simulink model "StampFly_IMU400"  (R2026b)
settings: Solver=FixedStepDiscrete  StopTime=inf  FixedStep=Official.Step
PostLoadFcn:
  | run(fullfile(fileparts(get_param('StampFly_IMU400','FileName')),'config','startup.m'));
InitFcn:
  | init_imu_flight;
undefined symbols (not defined in the file): Bottom, Official
libraries: slpidlib x7, simulink x4, mspfiltlib x1
(part 3 of 4)

== system StampFly_IMU400/SensorCorrection400/VerticalAcceleration/VerticalLowpass ==
  Input : Inport
  Dt : Inport  Port=2
  Reset : Inport  Port=3
  Enable : Inport  Port=4
  Denominator : Sum
  InputTerm : Product  Inputs=*/
  InputTimesDt : Product  Inputs=**
  PreviousFiltered : UnitDelay  InitialCondition=single(0)  SampleTime=.0025
  PreviousTerm : Product  Inputs=*/
  PreviousTimesT : Product  Inputs=**
  ResetPrevious : Switch  Criteria=u2 ~= 0  SaturateOnIntegerOverflow=off  InputSameDT=off
  TimeConstantS : Constant  Value=single(0.10000000000000001)
  UpdateOrHold : Switch  Criteria=u2 ~= 0  SaturateOnIntegerOverflow=off  InputSameDT=off
  UpdatedFiltered : Sum
  ZeroOnReset : Constant  Value=single(0)
  Filtered : Outport
  wires:
  Input/1 -> InputTimesDt/1
  Denominator/1 -> PreviousTerm/2, InputTerm/2
  InputTimesDt/1 -> InputTerm/1
  Dt/1 -> Denominator/2, InputTimesDt/2
  TimeConstantS/1 -> PreviousTimesT/2, Denominator/1
  Enable/1 -> UpdateOrHold/2
  InputTerm/1 -> UpdatedFiltered/2
  UpdatedFiltered/1 -> UpdateOrHold/1
  UpdateOrHold/1 -> PreviousFiltered/1, Filtered/1
  ZeroOnReset/1 -> ResetPrevious/1
  Reset/1 -> ResetPrevious/2
  PreviousFiltered/1 -> ResetPrevious/3
  ResetPrevious/1 -> UpdateOrHold/3, PreviousTimesT/1
  PreviousTimesT/1 -> PreviousTerm/1
  PreviousTerm/1 -> UpdatedFiltered/1

== system StampFly_IMU400/AttitudeAltitudeEstimation400/IMUAttitude400/FusionState/UpdateWhenReady ==
  Accel : Inport  PortDimensions=[1 3]
  Gyro : Inport  Port=2  PortDimensions=[1 3]
  Reset : ResetPort  DisableCoverage=on  ResetTriggerType=level
  IMU Filter : mspfiltlib/IMU Filter  DispRefFrame=NED  OrientationFormat=quaternion  DecimationFactor=1  InitialProcessNoise=IMUFlight.InitialProcessNoise  AccelerometerNoise=IMUFlight.AccelerometerNoise  GyroscopeNoise=IMUFlight.GyroscopeNoise  GyroscopeDriftNoise=IMUFlight.GyroscopeDriftNoise  LinearAccelerationNoise=IMUFlight.LinearAccelerationNoise  LinearAccelerationDecayFactor=IMUFlight.LinearAccelerationDecayFactor  SimulateUsing=Code generation
  Orientation : Outport  PortDimensions=[1 4]  InitialOutput=single([1 0 0 0])
  AngularVelocity : Outport  Port=2  PortDimensions=[1 3]  InitialOutput=single([0 0 0])
  wires:
  IMU Filter/2 -> AngularVelocity/1
  IMU Filter/1 -> Orientation/1
  Gyro/1 -> IMU Filter/2
  Accel/1 -> IMU Filter/1

== system StampFly_IMU400/FlightControl400/TakeoffHoverControl400/AltitudeControl400/AltitudePID ==
  Error : Inport
  Dt : Inport  Port=2
  Enable : Inport  Port=3
  Reset : Inport  Port=4
  PreviousError : Inport  Port=5
  EnabledPID : Subsystem
  UnusedPreviousError : Terminator
  Output : Outport
  wires:
  EnabledPID/1(Output) -> Output/1
  PreviousError/1 -> UnusedPreviousError/1
  Reset/1 -> EnabledPID/3(Reset)
  Dt/1 -> EnabledPID/2(Dt)
  Error/1 -> EnabledPID/1(Error)
  Enable/1 -> EnabledPID/Enable

== system StampFly_IMU400/FlightControl400/TakeoffHoverControl400/AltitudeControl400/VerticalSpeedPID ==
  Error : Inport
  Dt : Inport  Port=2
  Enable : Inport  Port=3
  Reset : Inport  Port=4
  PreviousError : Inport  Port=5
  EnabledPID : Subsystem
  UnusedPreviousError : Terminator
  Output : Outport
  wires:
  EnabledPID/1(Output) -> Output/1
  PreviousError/1 -> UnusedPreviousError/1
  Reset/1 -> EnabledPID/3(Reset)
  Dt/1 -> EnabledPID/2(Dt)
  Error/1 -> EnabledPID/1(Error)
  Enable/1 -> EnabledPID/Enable

== system StampFly_IMU400/FlightControl400/TakeoffHoverControl400/AttitudeControl400/PitchAnglePID ==
  Error : Inport
  Dt : Inport  Port=2
  Enable : Inport  Port=3
  Reset : Inport  Port=4
  PreviousError : Inport  Port=5
  EnabledPID : Subsystem
  UnusedPreviousError : Terminator
  Output : Outport
  wires:
  EnabledPID/1(Output) -> Output/1
  PreviousError/1 -> UnusedPreviousError/1
  Reset/1 -> EnabledPID/3(Reset)
  Dt/1 -> EnabledPID/2(Dt)
  Error/1 -> EnabledPID/1(Error)
  Enable/1 -> EnabledPID/Enable

== system StampFly_IMU400/FlightControl400/TakeoffHoverControl400/AttitudeControl400/RollAnglePID ==
  Error : Inport
  Dt : Inport  Port=2
  Enable : Inport  Port=3
  Reset : Inport  Port=4
  PreviousError : Inport  Port=5
  EnabledPID : Subsystem
  UnusedPreviousError : Terminator
  Output : Outport
  wires:
  EnabledPID/1(Output) -> Output/1
  PreviousError/1 -> UnusedPreviousError/1
  Reset/1 -> EnabledPID/3(Reset)
  Dt/1 -> EnabledPID/2(Dt)
  Error/1 -> EnabledPID/1(Error)
  Enable/1 -> EnabledPID/Enable

== system StampFly_IMU400/FlightControl400/TakeoffHoverControl400/BodyRateControl400/PitchRatePID ==
  Error : Inport
  Dt : Inport  Port=2
  Enable : Inport  Port=3
  Reset : Inport  Port=4
  PreviousError : Inport  Port=5
  EnabledPID : Subsystem
  UnusedPreviousError : Terminator
  Output : Outport
  wires:
  PreviousError/1 -> UnusedPreviousError/1
  Error/1 -> EnabledPID/1(Error)
  Enable/1 -> EnabledPID/Enable
  EnabledPID/1(Output) -> Output/1
  Reset/1 -> EnabledPID/3(Reset)
  Dt/1 -> EnabledPID/2(Dt)

== system StampFly_IMU400/FlightControl400/TakeoffHoverControl400/BodyRateControl400/RollRatePID ==
  Error : Inport
  Dt : Inport  Port=2
  Enable : Inport  Port=3
  Reset : Inport  Port=4
  PreviousError : Inport  Port=5
  EnabledPID : Subsystem
  UnusedPreviousError : Terminator
  Output : Outport
  wires:
  PreviousError/1 -> UnusedPreviousError/1
  Error/1 -> EnabledPID/1(Error)
  Enable/1 -> EnabledPID/Enable
  EnabledPID/1(Output) -> Output/1
  Reset/1 -> EnabledPID/3(Reset)
  Dt/1 -> EnabledPID/2(Dt)

== system StampFly_IMU400/FlightControl400/TakeoffHoverControl400/BodyRateControl400/YawRatePID ==
  Error : Inport
  Dt : Inport  Port=2
  Enable : Inport  Port=3
  Reset : Inport  Port=4
  PreviousError : Inport  Port=5
  EnabledPID : Subsystem
  UnusedPreviousError : Terminator
  Output : Outport
  wires:
  PreviousError/1 -> UnusedPreviousError/1
  Error/1 -> EnabledPID/1(Error)
  Enable/1 -> EnabledPID/Enable
  EnabledPID/1(Output) -> Output/1
  Reset/1 -> EnabledPID/3(Reset)
  Dt/1 -> EnabledPID/2(Dt)

== system StampFly_IMU400/FlightControl400/TakeoffHoverControl400/FlightCommand400/ControlGating400 ==
  CommandMode : Inport
  ModeContext : Inport  Port=2
  ThrustState : Inport  Port=3
  CommandModeFields : BusSelector  OutputSignals=RawThrust,ManualAltitude,AltitudeEnabled,ControlMode
  ControlContextBus : BusCreator  Inputs=5
  ControlEnableReset : MATLAB Function  Description=|  TreatAsAtomicUnit=on
      | 各 PID の実行条件を決める
      | 計算処理。飛行状態遷移はStateflowで管理。
  ModeContextFields : BusSelector  OutputSignals=FlightContext.Branch,Dt,Mode
  ThrustStateFields : BusSelector  OutputSignals=FilteredThrust,HeldThrust
  ThrustRequest : Outport
  ControlContext : Outport  Port=2
  wires:
  CommandModeFields/2 -> ControlEnableReset/2(arg_arg_manual)  "<ManualAltitude>"
  ThrustState/1 -> ThrustStateFields/1
  ControlEnableReset/5(arg_arg_angleEnable) -> ControlContextBus/4  "AngleEnabled"
  CommandMode/1 -> CommandModeFields/1
  CommandModeFields/4 -> ControlEnableReset/5(arg_arg_controlMode)  "<ControlMode>"
  ModeContext/1 -> ModeContextFields/1
  CommandModeFields/1 -> ControlEnableReset/1(arg_arg_raw)  "<RawThrust>"
  CommandModeFields/3 -> ControlEnableReset/3(arg_arg_auto)  "<AltitudeEnabled>"
  ModeContextFields/1 -> ControlEnableReset/4(arg_branch)  "<Branch>"
  ModeContextFields/2 -> ControlEnableReset/6(arg_arg_dt)  "<Dt>"
  ModeContextFields/3 -> ControlEnableReset/9(arg_arg_mode)  "<Mode>"
  ThrustStateFields/1 -> ControlEnableReset/7(arg_arg_oldFilter)  "<FilteredThrust>"
  ThrustStateFields/2 -> ControlEnableReset/8(arg_arg_lastThrust)  "<HeldThrust>"
  ControlEnableReset/1(arg_arg_command) -> ThrustRequest/1  "ThrustRequest"
  ControlEnableReset/2(arg_arg_run) -> ControlContextBus/1  "Run"
  ControlEnableReset/3(arg_arg_reset) -> ControlContextBus/2  "Reset"
  ControlEnableReset/4(arg_arg_altEnable) -> ControlContextBus/3  "AltitudeEnabled"
  ControlEnableReset/6(arg_arg_velEnable) -> ControlContextBus/5  "VelocityEnabled"
  ControlContextBus/1 -> ControlContext/1  "ControlContext"

== system StampFly_IMU400/FlightControl400/TakeoffHoverControl400/FlightCommand400/UnusedStickFields ==
  Sticks : Inport
  StickFields : Demux  Outputs=6
  UnusedStick{1..4,6} (5 alike) : Terminator
  UnusedStickMode : Terminator
  wires:
  StickFields/6 -> UnusedStick6/1
  StickFields/2 -> UnusedStick2/1
  Sticks/1 -> StickFields/1
  StickFields/5 -> UnusedStickMode/1
  StickFields/1 -> UnusedStick1/1
  StickFields/3 -> UnusedStick3/1
  StickFields/4 -> UnusedStick4/1

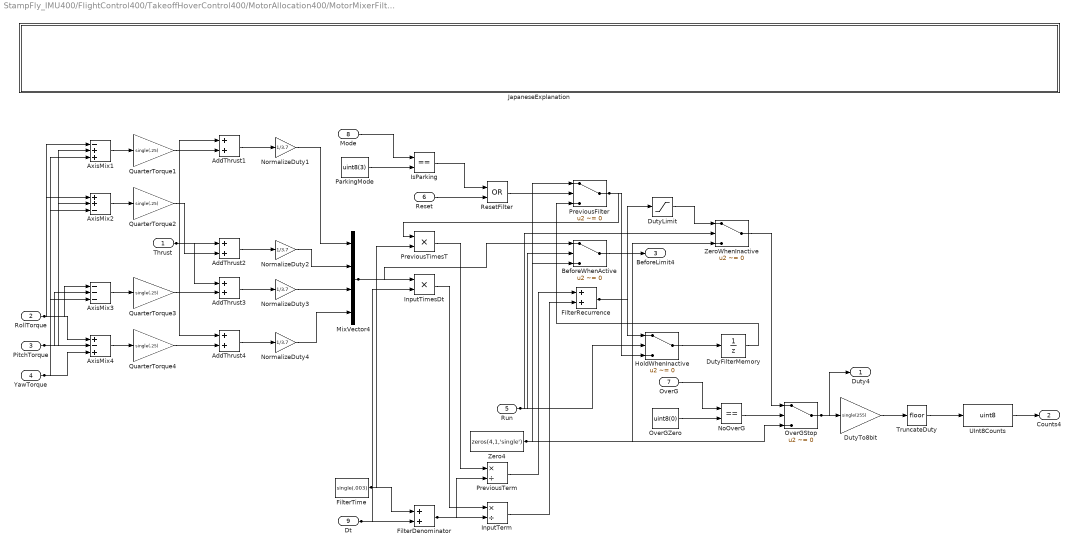
== system StampFly_IMU400/FlightControl400/TakeoffHoverControl400/MotorAllocation400/MotorMixerFilter8bit ==
  Thrust : Inport
  RollTorque : Inport  Port=2
  PitchTorque : Inport  Port=3
  YawTorque : Inport  Port=4
  Run : Inport  Port=5
  Reset : Inport  Port=6
  OverG : Inport  Port=7
  Mode : Inport  Port=8
  Dt : Inport  Port=9
  AddThrust{1..4} (4 alike) : Sum
  AxisMix1 : Sum  Inputs=-++
  AxisMix2 : Sum  Inputs=++-
  AxisMix3 : Sum  Inputs=---
  AxisMix4 : Sum  Inputs=+-+
  BeforeWhenActive : Switch  Criteria=u2 ~= 0  SaturateOnIntegerOverflow=off  InputSameDT=off
  DutyFilterMemory : UnitDelay  InitialCondition=zeros(4,1,'single')  SampleTime=Official.Step
  DutyLimit : Saturate  UpperLimit=single(.95)  LowerLimit=single(0)
  DutyTo8bit : Gain  Gain=single(255)
  FilterDenominator : Sum
  FilterRecurrence : Sum
  FilterTime : Constant  Value=single(.003)
  HoldWhenInactive : Switch  Criteria=u2 ~= 0  SaturateOnIntegerOverflow=off  InputSameDT=off
  InputTerm : Product  Inputs=*/
  InputTimesDt : Product
  IsParking : RelationalOperator  Operator===  OutDataTypeStr=boolean  RndMeth=Simplest  InputSameDT=off
  JapaneseExplanation : Subsystem  Description=推力と3軸トルクを4モーターへ配分。元のフィルター、Duty上限0.95、8 bit量子化を維持しています。
      mask Display: disp('推力と3軸トルクを4モーターへ配分。元のフィルター、Duty上限0.95、8 bit量子化を維持しています。')
  MixVector4 : Mux
  NoOverG : RelationalOperator  Operator===  OutDataTypeStr=boolean  RndMeth=Simplest  InputSameDT=off
  NormalizeDuty{1..4} (4 alike) : Gain  Gain=1/3.7  OutDataTypeStr=single
  OverGStop : Switch  Criteria=u2 ~= 0  SaturateOnIntegerOverflow=off  InputSameDT=off
  OverGZero : Constant  Value=uint8(0)
  ParkingMode : Constant  Value=uint8(3)
  PreviousFilter : Switch  Criteria=u2 ~= 0  SaturateOnIntegerOverflow=off  InputSameDT=off
  PreviousTerm : Product  Inputs=*/
  PreviousTimesT : Product
  QuarterTorque{1..4} (4 alike) : Gain  Gain=single(.25)
  ResetFilter : Logic  Operator=OR  AllPortsSameDT=off  OutDataTypeStr=boolean
  TruncateDuty : Rounding
  UInt8Counts : DataTypeConversion  OutDataTypeStr=uint8  SaturateOnIntegerOverflow=off  RndMeth=Floor
  Zero4 : Constant  Value=zeros(4,1,'single')
  ZeroWhenInactive : Switch  Criteria=u2 ~= 0  SaturateOnIntegerOverflow=off  InputSameDT=off
  Duty4 : Outport
  Counts4 : Outport  Port=2
  BeforeLimit4 : Outport  Port=3
  wires:
  YawTorque/1 -> AxisMix1/3, AxisMix2/3, AxisMix3/3, AxisMix4/3
  RollTorque/1 -> AxisMix3/1, AxisMix4/1, AxisMix1/1, AxisMix2/1
  PitchTorque/1 -> AxisMix4/2, AxisMix3/2, AxisMix2/2, AxisMix1/2
  MixVector4/1 -> InputTimesDt/1, BeforeWhenActive/1
  AxisMix1/1 -> QuarterTorque1/1
  QuarterTorque1/1 -> AddThrust1/2
  AxisMix2/1 -> QuarterTorque2/1
  NormalizeDuty2/1 -> MixVector4/2
  AxisMix3/1 -> QuarterTorque3/1
  QuarterTorque3/1 -> AddThrust3/2
  AxisMix4/1 -> QuarterTorque4/1
  QuarterTorque2/1 -> AddThrust2/2
  ZeroWhenInactive/1 -> OverGStop/1
  Thrust/1 -> AddThrust1/1, AddThrust2/1, AddThrust4/1, AddThrust3/1
  QuarterTorque4/1 -> AddThrust4/2
  AddThrust1/1 -> NormalizeDuty1/1
  AddThrust2/1 -> NormalizeDuty2/1
  AddThrust3/1 -> NormalizeDuty3/1
  AddThrust4/1 -> NormalizeDuty4/1
  NormalizeDuty1/1 -> MixVector4/1
  HoldWhenInactive/1 -> DutyFilterMemory/1
  NormalizeDuty3/1 -> MixVector4/3
  NormalizeDuty4/1 -> MixVector4/4
  Mode/1 -> IsParking/1
  TruncateDuty/1 -> UInt8Counts/1
  IsParking/1 -> ResetFilter/1
  ParkingMode/1 -> IsParking/2
  FilterTime/1 -> FilterDenominator/1, PreviousTimesT/2
  Dt/1 -> FilterDenominator/2, InputTimesDt/2
  Reset/1 -> ResetFilter/2
  FilterRecurrence/1 -> HoldWhenInactive/1, DutyLimit/1
  PreviousTimesT/1 -> PreviousTerm/1
  OverGStop/1 -> Duty4/1, DutyTo8bit/1
  BeforeWhenActive/1 -> BeforeLimit4/1
  InputTimesDt/1 -> InputTerm/1
  PreviousTerm/1 -> FilterRecurrence/1
  FilterDenominator/1 -> PreviousTerm/2, InputTerm/2
  ResetFilter/1 -> PreviousFilter/2
  Run/1 -> ZeroWhenInactive/2, HoldWhenInactive/2, BeforeWhenActive/2
  Zero4/1 -> ZeroWhenInactive/3, OverGStop/3, PreviousFilter/1, BeforeWhenActive/3
  InputTerm/1 -> FilterRecurrence/2
  DutyTo8bit/1 -> TruncateDuty/1
  PreviousFilter/1 -> PreviousTimesT/1, HoldWhenInactive/3
  DutyLimit/1 -> ZeroWhenInactive/1
  OverG/1 -> NoOverG/1
  OverGZero/1 -> NoOverG/2
  DutyFilterMemory/1 -> PreviousFilter/3
  NoOverG/1 -> OverGStop/2
  UInt8Counts/1 -> Counts4/1

== system StampFly_IMU400/FlightControl400/TakeoffHoverControl400/AltitudeControl400/AltitudePID/EnabledPID ==
  Error : Inport
  Dt : Inport  Port=2
  Reset : Inport  Port=3
  Enable : EnablePort
  DedicatedPID : slpidlib/PID Controller  Description=飛行比較用の専用PID。Ideal形式、台形積分・微分フィルター、実測Dt、単精度。  Controller=PID  Form=Ideal  TimeDomain=Discrete-time  UseExternalTs=on  SampleTime=.0025  IntegratorMethod=Trapezoidal  FilterMethod=Trapezoidal  ControllerParametersSource=internal  P=single(0.37999999523162842)  I=single(1)/single(10)  UseKiTs=off  D=single(0.5)  UseExternalDerivativeSource=off  N=single(1)/(single(0.125)*single(0.5))  UseFilter=on  TunerSelectOption=Transfer Function Based (PID Tuner App)  InitialConditionSource=external  InitialConditionForIntegrator=0  InitialConditionForFilter=0  DifferentiatorICPrevScaledInput=0  ExternalReset=level  TrackingMode=off  Kt=1  LimitOutput=off  SatLimitsSource=internal  UpperSaturationLimit=inf  LowerSaturationLimit=-inf  LinearizeAsGain=off  AntiWindupMode=none  Kb=1  LimitIntegrator=on  UpperIntegratorSaturationLimit=single(30000)  LowerIntegratorSaturationLimit=single(-30000)  PGainOutDataTypeStr=single  PProdOutDataTypeStr=single  POutMin=[]  POutMax=[]  IGainOutDataTypeStr=single  IProdOutDataTypeStr=single  IOutMin=[]  IOutMax=[]  DGainOutDataTypeStr=single  DProdOutDataTypeStr=single  DOutMin=[]  DOutMax=[]  NGainOutDataTypeStr=single  NProdOutDataTypeStr=single  NOutMin=[]  NOutMax=[]  SumOutDataTypeStr=single  SumOutMin=[]  SumOutMax=[]  SaturationOutDataTypeStr=single  SaturationOutMin=[]  SaturationOutMax=[]  PParamDataTypeStr=single  PParamMin=[]  PParamMax=[]  IParamDataTypeStr=single  IParamMin=[]  IParamMax=[]  DParamDataTypeStr=single  DParamMin=[]  DParamMax=[]  NParamDataTypeStr=single  NParamMin=[]  NParamMax=[]  KbParamDataTypeStr=single  KbParamMin=[]  KbParamMax=[]  KtParamDataTypeStr=single  KtParamMin=[]  KtParamMax=[]  KbOutDataTypeStr=single  KbOutMin=[]  KbOutMax=[]  KtOutDataTypeStr=single  KtOutMin=[]  KtOutMax=[]  IntegratorOutDataTypeStr=single  IntegratorOutMin=[]  IntegratorOutMax=[]  FilterOutDataTypeStr=single  FilterOutMin=[]  FilterOutMax=[]  SumI1OutDataTypeStr=single  SumI1OutMin=[]  SumI1OutMax=[]  SumI2OutDataTypeStr=single  SumI2OutMin=[]  SumI2OutMax=[]  SumI3OutDataTypeStr=single  SumI3OutMin=[]  SumI3OutMax=[]  SumI4OutDataTypeStr=single  SumI4OutMin=[]  SumI4OutMax=[]  SumDOutDataTypeStr=single  SumDOutMin=[]  SumDOutMax=[]  SumAccumDataTypeStr=single  SumI1AccumDataTypeStr=single  SumI2AccumDataTypeStr=single  SumI3AccumDataTypeStr=single  SumI4AccumDataTypeStr=single  SumDAccumDataTypeStr=single  DifferentiatorOutDataTypeStr=single  DifferentiatorOutMin=[]  DifferentiatorOutMax=[]  FilterDiffOutCoefMin=[]  FilterDiffOutCoefMax=[]  ReciprocalOutDataTypeStr=single  ReciprocalOutMin=[]  ReciprocalOutMax=[]  SumDenOutDataTypeStr=single  SumDenOutMin=[]  SumDenOutMax=[]  SumNumOutDataTypeStr=single  SumNumOutMin=[]  SumNumOutMax=[]  SumDenAccumDataTypeStr=single  SumNumAccumDataTypeStr=single  DivideOutDataTypeStr=single  DivideOutMin=[]  DivideOutMax=[]  UdiffTsProdOutDataTypeStr=single  UdiffTsProdOutMin=[]  UdiffTsProdOutMax=[]  NTsProdOutDataTypeStr=single  NTsProdOutMin=[]  NTsProdOutMax=[]  UintegralTsProdOutDataTypeStr=single  UintegralTsProdOutMin=[]  UintegralTsProdOutMax=[]  UngainTsProdOutDataTypeStr=single  UngainTsProdOutMin=[]  UngainTsProdOutMax=[]  ClampingZeroOutDataTypeStr=single  ClampingZeroOutMin=[]  ClampingZeroOutMax=[]  FilterDenConstantOutDataTypeStr=single  FilterDenConstantOutMin=[]  FilterDenConstantOutMax=[]  PCopyOutDataTypeStr=single  PCopyOutMin=[]  PCopyOutMax=[]  NCopyOutDataTypeStr=single  NCopyOutMin=[]  NCopyOutMax=[]  IntegratorContinuousStateAttributes=''  IntegratorStateMustResolveToSignalObject=off  IntegratorRTWStateStorageClass=Auto  FilterContinuousStateAttributes=''  FilterStateMustResolveToSignalObject=off  FilterRTWStateStorageClass=Auto  ParallelPVariant=Passthrough  IdealPVariant=InternalParameters  IVariant=InternalParameters  DVariant=InternalParameters  IntegratorVariant=Discrete  SatVariant=Disabled  AWVariant=Passthrough  PCopyVariant=Disabled  TRVariant=Disabled  FdbkBlocksVariant=Forward  IdealPFdbkVariant=Disabled  SatFdbkVariant=Disabled  DerivativeFilterVariant=TrapezoidalFilter  NVariant=InternalParameters  NCopyVariant=InternalParameters  FilterICVariant=ExternalICs  IntegratorICVariant=ExternalICs  ExternalResetVariant=ExternalReset  TRSumVariant=Passthrough  SumFdbkVariant=Disabled  SumVariant=Sum_PID  TsampFilterVariant=ExternalTs  TsampNgainVariant=Passthrough  TsampIntegralVariant=ExternalTs  ExternalSaturationOutDataTypeStr=Inherit: Same as second input  DerivativeSourceVariant=ErrorSignal  PreIntVariant=InternalPreInt
      settings: LibrarySourceBlock=simulink/Discrete/Discrete PID Controller
  ZeroInitialCondition : Constant  Value=single(0)
  Output : Outport
  wires:
  Dt/1 -> DedicatedPID/5
  Reset/1 -> DedicatedPID/2
  Error/1 -> DedicatedPID/1
  DedicatedPID/1 -> Output/1
  ZeroInitialCondition/1 -> DedicatedPID/3, DedicatedPID/4

== system StampFly_IMU400/FlightControl400/TakeoffHoverControl400/AltitudeControl400/VerticalSpeedPID/EnabledPID ==
  Error : Inport
  Dt : Inport  Port=2
  Reset : Inport  Port=3
  Enable : EnablePort
  DedicatedPID : slpidlib/PID Controller  Description=飛行比較用の専用PID。Ideal形式、台形積分・微分フィルター、実測Dt、単精度。  Controller=PID  Form=Ideal  TimeDomain=Discrete-time  UseExternalTs=on  SampleTime=.0025  IntegratorMethod=Trapezoidal  FilterMethod=Trapezoidal  ControllerParametersSource=internal  P=single(0.079999998211860657)  I=single(1)/single(0.94999998807907104)  UseKiTs=off  D=single(0.079999998211860657)  UseExternalDerivativeSource=off  N=single(1)/(single(0.125)*single(0.079999998211860657))  UseFilter=on  TunerSelectOption=Transfer Function Based (PID Tuner App)  InitialConditionSource=external  InitialConditionForIntegrator=0  InitialConditionForFilter=0  DifferentiatorICPrevScaledInput=0  ExternalReset=level  TrackingMode=off  Kt=1  LimitOutput=off  SatLimitsSource=internal  UpperSaturationLimit=inf  LowerSaturationLimit=-inf  LinearizeAsGain=off  AntiWindupMode=none  Kb=1  LimitIntegrator=on  UpperIntegratorSaturationLimit=single(30000)  LowerIntegratorSaturationLimit=single(-30000)  PGainOutDataTypeStr=single  PProdOutDataTypeStr=single  POutMin=[]  POutMax=[]  IGainOutDataTypeStr=single  IProdOutDataTypeStr=single  IOutMin=[]  IOutMax=[]  DGainOutDataTypeStr=single  DProdOutDataTypeStr=single  DOutMin=[]  DOutMax=[]  NGainOutDataTypeStr=single  NProdOutDataTypeStr=single  NOutMin=[]  NOutMax=[]  SumOutDataTypeStr=single  SumOutMin=[]  SumOutMax=[]  SaturationOutDataTypeStr=single  SaturationOutMin=[]  SaturationOutMax=[]  PParamDataTypeStr=single  PParamMin=[]  PParamMax=[]  IParamDataTypeStr=single  IParamMin=[]  IParamMax=[]  DParamDataTypeStr=single  DParamMin=[]  DParamMax=[]  NParamDataTypeStr=single  NParamMin=[]  NParamMax=[]  KbParamDataTypeStr=single  KbParamMin=[]  KbParamMax=[]  KtParamDataTypeStr=single  KtParamMin=[]  KtParamMax=[]  KbOutDataTypeStr=single  KbOutMin=[]  KbOutMax=[]  KtOutDataTypeStr=single  KtOutMin=[]  KtOutMax=[]  IntegratorOutDataTypeStr=single  IntegratorOutMin=[]  IntegratorOutMax=[]  FilterOutDataTypeStr=single  FilterOutMin=[]  FilterOutMax=[]  SumI1OutDataTypeStr=single  SumI1OutMin=[]  SumI1OutMax=[]  SumI2OutDataTypeStr=single  SumI2OutMin=[]  SumI2OutMax=[]  SumI3OutDataTypeStr=single  SumI3OutMin=[]  SumI3OutMax=[]  SumI4OutDataTypeStr=single  SumI4OutMin=[]  SumI4OutMax=[]  SumDOutDataTypeStr=single  SumDOutMin=[]  SumDOutMax=[]  SumAccumDataTypeStr=single  SumI1AccumDataTypeStr=single  SumI2AccumDataTypeStr=single  SumI3AccumDataTypeStr=single  SumI4AccumDataTypeStr=single  SumDAccumDataTypeStr=single  DifferentiatorOutDataTypeStr=single  DifferentiatorOutMin=[]  DifferentiatorOutMax=[]  FilterDiffOutCoefMin=[]  FilterDiffOutCoefMax=[]  ReciprocalOutDataTypeStr=single  ReciprocalOutMin=[]  ReciprocalOutMax=[]  SumDenOutDataTypeStr=single  SumDenOutMin=[]  SumDenOutMax=[]  SumNumOutDataTypeStr=single  SumNumOutMin=[]  SumNumOutMax=[]  SumDenAccumDataTypeStr=single  SumNumAccumDataTypeStr=single  DivideOutDataTypeStr=single  DivideOutMin=[]  DivideOutMax=[]  UdiffTsProdOutDataTypeStr=single  UdiffTsProdOutMin=[]  UdiffTsProdOutMax=[]  NTsProdOutDataTypeStr=single  NTsProdOutMin=[]  NTsProdOutMax=[]  UintegralTsProdOutDataTypeStr=single  UintegralTsProdOutMin=[]  UintegralTsProdOutMax=[]  UngainTsProdOutDataTypeStr=single  UngainTsProdOutMin=[]  UngainTsProdOutMax=[]  ClampingZeroOutDataTypeStr=single  ClampingZeroOutMin=[]  ClampingZeroOutMax=[]  FilterDenConstantOutDataTypeStr=single  FilterDenConstantOutMin=[]  FilterDenConstantOutMax=[]  PCopyOutDataTypeStr=single  PCopyOutMin=[]  PCopyOutMax=[]  NCopyOutDataTypeStr=single  NCopyOutMin=[]  NCopyOutMax=[]  IntegratorContinuousStateAttributes=''  IntegratorStateMustResolveToSignalObject=off  IntegratorRTWStateStorageClass=Auto  FilterContinuousStateAttributes=''  FilterStateMustResolveToSignalObject=off  FilterRTWStateStorageClass=Auto  ParallelPVariant=Passthrough  IdealPVariant=InternalParameters  IVariant=InternalParameters  DVariant=InternalParameters  IntegratorVariant=Discrete  SatVariant=Disabled  AWVariant=Passthrough  PCopyVariant=Disabled  TRVariant=Disabled  FdbkBlocksVariant=Forward  IdealPFdbkVariant=Disabled  SatFdbkVariant=Disabled  DerivativeFilterVariant=TrapezoidalFilter  NVariant=InternalParameters  NCopyVariant=InternalParameters  FilterICVariant=ExternalICs  IntegratorICVariant=ExternalICs  ExternalResetVariant=ExternalReset  TRSumVariant=Passthrough  SumFdbkVariant=Disabled  SumVariant=Sum_PID  TsampFilterVariant=ExternalTs  TsampNgainVariant=Passthrough  TsampIntegralVariant=ExternalTs  ExternalSaturationOutDataTypeStr=Inherit: Same as second input  DerivativeSourceVariant=ErrorSignal  PreIntVariant=InternalPreInt
      settings: LibrarySourceBlock=simulink/Discrete/Discrete PID Controller
  ZeroInitialCondition : Constant  Value=single(0)
  Output : Outport
  wires:
  DedicatedPID/1 -> Output/1
  Dt/1 -> DedicatedPID/5
  ZeroInitialCondition/1 -> DedicatedPID/3, DedicatedPID/4
  Reset/1 -> DedicatedPID/2
  Error/1 -> DedicatedPID/1

== system StampFly_IMU400/FlightControl400/TakeoffHoverControl400/AttitudeControl400/PitchAnglePID/EnabledPID ==
  Error : Inport
  Dt : Inport  Port=2
  Reset : Inport  Port=3
  Enable : EnablePort
  DedicatedPID : slpidlib/PID Controller  Description=飛行比較用の専用PID。Ideal形式、台形積分・微分フィルター、実測Dt、単精度。  Controller=PID  Form=Ideal  TimeDomain=Discrete-time  UseExternalTs=on  SampleTime=.0025  IntegratorMethod=Trapezoidal  FilterMethod=Trapezoidal  ControllerParametersSource=internal  P=single(5)  I=single(1)/single(4)  UseKiTs=off  D=single(0.039999999105930328)  UseExternalDerivativeSource=off  N=single(1)/(single(0.125)*single(0.039999999105930328))  UseFilter=on  TunerSelectOption=Transfer Function Based (PID Tuner App)  InitialConditionSource=external  InitialConditionForIntegrator=0  InitialConditionForFilter=0  DifferentiatorICPrevScaledInput=0  ExternalReset=level  TrackingMode=off  Kt=1  LimitOutput=off  SatLimitsSource=internal  UpperSaturationLimit=inf  LowerSaturationLimit=-inf  LinearizeAsGain=off  AntiWindupMode=none  Kb=1  LimitIntegrator=on  UpperIntegratorSaturationLimit=single(30000)  LowerIntegratorSaturationLimit=single(-30000)  PGainOutDataTypeStr=single  PProdOutDataTypeStr=single  POutMin=[]  POutMax=[]  IGainOutDataTypeStr=single  IProdOutDataTypeStr=single  IOutMin=[]  IOutMax=[]  DGainOutDataTypeStr=single  DProdOutDataTypeStr=single  DOutMin=[]  DOutMax=[]  NGainOutDataTypeStr=single  NProdOutDataTypeStr=single  NOutMin=[]  NOutMax=[]  SumOutDataTypeStr=single  SumOutMin=[]  SumOutMax=[]  SaturationOutDataTypeStr=single  SaturationOutMin=[]  SaturationOutMax=[]  PParamDataTypeStr=single  PParamMin=[]  PParamMax=[]  IParamDataTypeStr=single  IParamMin=[]  IParamMax=[]  DParamDataTypeStr=single  DParamMin=[]  DParamMax=[]  NParamDataTypeStr=single  NParamMin=[]  NParamMax=[]  KbParamDataTypeStr=single  KbParamMin=[]  KbParamMax=[]  KtParamDataTypeStr=single  KtParamMin=[]  KtParamMax=[]  KbOutDataTypeStr=single  KbOutMin=[]  KbOutMax=[]  KtOutDataTypeStr=single  KtOutMin=[]  KtOutMax=[]  IntegratorOutDataTypeStr=single  IntegratorOutMin=[]  IntegratorOutMax=[]  FilterOutDataTypeStr=single  FilterOutMin=[]  FilterOutMax=[]  SumI1OutDataTypeStr=single  SumI1OutMin=[]  SumI1OutMax=[]  SumI2OutDataTypeStr=single  SumI2OutMin=[]  SumI2OutMax=[]  SumI3OutDataTypeStr=single  SumI3OutMin=[]  SumI3OutMax=[]  SumI4OutDataTypeStr=single  SumI4OutMin=[]  SumI4OutMax=[]  SumDOutDataTypeStr=single  SumDOutMin=[]  SumDOutMax=[]  SumAccumDataTypeStr=single  SumI1AccumDataTypeStr=single  SumI2AccumDataTypeStr=single  SumI3AccumDataTypeStr=single  SumI4AccumDataTypeStr=single  SumDAccumDataTypeStr=single  DifferentiatorOutDataTypeStr=single  DifferentiatorOutMin=[]  DifferentiatorOutMax=[]  FilterDiffOutCoefMin=[]  FilterDiffOutCoefMax=[]  ReciprocalOutDataTypeStr=single  ReciprocalOutMin=[]  ReciprocalOutMax=[]  SumDenOutDataTypeStr=single  SumDenOutMin=[]  SumDenOutMax=[]  SumNumOutDataTypeStr=single  SumNumOutMin=[]  SumNumOutMax=[]  SumDenAccumDataTypeStr=single  SumNumAccumDataTypeStr=single  DivideOutDataTypeStr=single  DivideOutMin=[]  DivideOutMax=[]  UdiffTsProdOutDataTypeStr=single  UdiffTsProdOutMin=[]  UdiffTsProdOutMax=[]  NTsProdOutDataTypeStr=single  NTsProdOutMin=[]  NTsProdOutMax=[]  UintegralTsProdOutDataTypeStr=single  UintegralTsProdOutMin=[]  UintegralTsProdOutMax=[]  UngainTsProdOutDataTypeStr=single  UngainTsProdOutMin=[]  UngainTsProdOutMax=[]  ClampingZeroOutDataTypeStr=single  ClampingZeroOutMin=[]  ClampingZeroOutMax=[]  FilterDenConstantOutDataTypeStr=single  FilterDenConstantOutMin=[]  FilterDenConstantOutMax=[]  PCopyOutDataTypeStr=single  PCopyOutMin=[]  PCopyOutMax=[]  NCopyOutDataTypeStr=single  NCopyOutMin=[]  NCopyOutMax=[]  IntegratorContinuousStateAttributes=''  IntegratorStateMustResolveToSignalObject=off  IntegratorRTWStateStorageClass=Auto  FilterContinuousStateAttributes=''  FilterStateMustResolveToSignalObject=off  FilterRTWStateStorageClass=Auto  ParallelPVariant=Passthrough  IdealPVariant=InternalParameters  IVariant=InternalParameters  DVariant=InternalParameters  IntegratorVariant=Discrete  SatVariant=Disabled  AWVariant=Passthrough  PCopyVariant=Disabled  TRVariant=Disabled  FdbkBlocksVariant=Forward  IdealPFdbkVariant=Disabled  SatFdbkVariant=Disabled  DerivativeFilterVariant=TrapezoidalFilter  NVariant=InternalParameters  NCopyVariant=InternalParameters  FilterICVariant=ExternalICs  IntegratorICVariant=ExternalICs  ExternalResetVariant=ExternalReset  TRSumVariant=Passthrough  SumFdbkVariant=Disabled  SumVariant=Sum_PID  TsampFilterVariant=ExternalTs  TsampNgainVariant=Passthrough  TsampIntegralVariant=ExternalTs  ExternalSaturationOutDataTypeStr=Inherit: Same as second input  DerivativeSourceVariant=ErrorSignal  PreIntVariant=InternalPreInt
      settings: LibrarySourceBlock=simulink/Discrete/Discrete PID Controller
  ZeroInitialCondition : Constant  Value=single(0)
  Output : Outport
  wires:
  Dt/1 -> DedicatedPID/5
  Error/1 -> DedicatedPID/1
  DedicatedPID/1 -> Output/1
  ZeroInitialCondition/1 -> DedicatedPID/3, DedicatedPID/4
  Reset/1 -> DedicatedPID/2

== system StampFly_IMU400/FlightControl400/TakeoffHoverControl400/AttitudeControl400/RollAnglePID/EnabledPID ==
  Error : Inport
  Dt : Inport  Port=2
  Reset : Inport  Port=3
  Enable : EnablePort
  DedicatedPID : slpidlib/PID Controller  Description=飛行比較用の専用PID。Ideal形式、台形積分・微分フィルター、実測Dt、単精度。  Controller=PID  Form=Ideal  TimeDomain=Discrete-time  UseExternalTs=on  SampleTime=.0025  IntegratorMethod=Trapezoidal  FilterMethod=Trapezoidal  ControllerParametersSource=internal  P=single(5)  I=single(1)/single(4)  UseKiTs=off  D=single(0.039999999105930328)  UseExternalDerivativeSource=off  N=single(1)/(single(0.125)*single(0.039999999105930328))  UseFilter=on  TunerSelectOption=Transfer Function Based (PID Tuner App)  InitialConditionSource=external  InitialConditionForIntegrator=0  InitialConditionForFilter=0  DifferentiatorICPrevScaledInput=0  ExternalReset=level  TrackingMode=off  Kt=1  LimitOutput=off  SatLimitsSource=internal  UpperSaturationLimit=inf  LowerSaturationLimit=-inf  LinearizeAsGain=off  AntiWindupMode=none  Kb=1  LimitIntegrator=on  UpperIntegratorSaturationLimit=single(30000)  LowerIntegratorSaturationLimit=single(-30000)  PGainOutDataTypeStr=single  PProdOutDataTypeStr=single  POutMin=[]  POutMax=[]  IGainOutDataTypeStr=single  IProdOutDataTypeStr=single  IOutMin=[]  IOutMax=[]  DGainOutDataTypeStr=single  DProdOutDataTypeStr=single  DOutMin=[]  DOutMax=[]  NGainOutDataTypeStr=single  NProdOutDataTypeStr=single  NOutMin=[]  NOutMax=[]  SumOutDataTypeStr=single  SumOutMin=[]  SumOutMax=[]  SaturationOutDataTypeStr=single  SaturationOutMin=[]  SaturationOutMax=[]  PParamDataTypeStr=single  PParamMin=[]  PParamMax=[]  IParamDataTypeStr=single  IParamMin=[]  IParamMax=[]  DParamDataTypeStr=single  DParamMin=[]  DParamMax=[]  NParamDataTypeStr=single  NParamMin=[]  NParamMax=[]  KbParamDataTypeStr=single  KbParamMin=[]  KbParamMax=[]  KtParamDataTypeStr=single  KtParamMin=[]  KtParamMax=[]  KbOutDataTypeStr=single  KbOutMin=[]  KbOutMax=[]  KtOutDataTypeStr=single  KtOutMin=[]  KtOutMax=[]  IntegratorOutDataTypeStr=single  IntegratorOutMin=[]  IntegratorOutMax=[]  FilterOutDataTypeStr=single  FilterOutMin=[]  FilterOutMax=[]  SumI1OutDataTypeStr=single  SumI1OutMin=[]  SumI1OutMax=[]  SumI2OutDataTypeStr=single  SumI2OutMin=[]  SumI2OutMax=[]  SumI3OutDataTypeStr=single  SumI3OutMin=[]  SumI3OutMax=[]  SumI4OutDataTypeStr=single  SumI4OutMin=[]  SumI4OutMax=[]  SumDOutDataTypeStr=single  SumDOutMin=[]  SumDOutMax=[]  SumAccumDataTypeStr=single  SumI1AccumDataTypeStr=single  SumI2AccumDataTypeStr=single  SumI3AccumDataTypeStr=single  SumI4AccumDataTypeStr=single  SumDAccumDataTypeStr=single  DifferentiatorOutDataTypeStr=single  DifferentiatorOutMin=[]  DifferentiatorOutMax=[]  FilterDiffOutCoefMin=[]  FilterDiffOutCoefMax=[]  ReciprocalOutDataTypeStr=single  ReciprocalOutMin=[]  ReciprocalOutMax=[]  SumDenOutDataTypeStr=single  SumDenOutMin=[]  SumDenOutMax=[]  SumNumOutDataTypeStr=single  SumNumOutMin=[]  SumNumOutMax=[]  SumDenAccumDataTypeStr=single  SumNumAccumDataTypeStr=single  DivideOutDataTypeStr=single  DivideOutMin=[]  DivideOutMax=[]  UdiffTsProdOutDataTypeStr=single  UdiffTsProdOutMin=[]  UdiffTsProdOutMax=[]  NTsProdOutDataTypeStr=single  NTsProdOutMin=[]  NTsProdOutMax=[]  UintegralTsProdOutDataTypeStr=single  UintegralTsProdOutMin=[]  UintegralTsProdOutMax=[]  UngainTsProdOutDataTypeStr=single  UngainTsProdOutMin=[]  UngainTsProdOutMax=[]  ClampingZeroOutDataTypeStr=single  ClampingZeroOutMin=[]  ClampingZeroOutMax=[]  FilterDenConstantOutDataTypeStr=single  FilterDenConstantOutMin=[]  FilterDenConstantOutMax=[]  PCopyOutDataTypeStr=single  PCopyOutMin=[]  PCopyOutMax=[]  NCopyOutDataTypeStr=single  NCopyOutMin=[]  NCopyOutMax=[]  IntegratorContinuousStateAttributes=''  IntegratorStateMustResolveToSignalObject=off  IntegratorRTWStateStorageClass=Auto  FilterContinuousStateAttributes=''  FilterStateMustResolveToSignalObject=off  FilterRTWStateStorageClass=Auto  ParallelPVariant=Passthrough  IdealPVariant=InternalParameters  IVariant=InternalParameters  DVariant=InternalParameters  IntegratorVariant=Discrete  SatVariant=Disabled  AWVariant=Passthrough  PCopyVariant=Disabled  TRVariant=Disabled  FdbkBlocksVariant=Forward  IdealPFdbkVariant=Disabled  SatFdbkVariant=Disabled  DerivativeFilterVariant=TrapezoidalFilter  NVariant=InternalParameters  NCopyVariant=InternalParameters  FilterICVariant=ExternalICs  IntegratorICVariant=ExternalICs  ExternalResetVariant=ExternalReset  TRSumVariant=Passthrough  SumFdbkVariant=Disabled  SumVariant=Sum_PID  TsampFilterVariant=ExternalTs  TsampNgainVariant=Passthrough  TsampIntegralVariant=ExternalTs  ExternalSaturationOutDataTypeStr=Inherit: Same as second input  DerivativeSourceVariant=ErrorSignal  PreIntVariant=InternalPreInt
      settings: LibrarySourceBlock=simulink/Discrete/Discrete PID Controller
  ZeroInitialCondition : Constant  Value=single(0)
  Output : Outport
  wires:
  Error/1 -> DedicatedPID/1
  DedicatedPID/1 -> Output/1
  Reset/1 -> DedicatedPID/2
  Dt/1 -> DedicatedPID/5
  ZeroInitialCondition/1 -> DedicatedPID/4, DedicatedPID/3

== system StampFly_IMU400/FlightControl400/TakeoffHoverControl400/BodyRateControl400/PitchRatePID/EnabledPID ==
  Error : Inport
  Dt : Inport  Port=2
  Reset : Inport  Port=3
  Enable : EnablePort
  DedicatedPID : slpidlib/PID Controller  Description=飛行比較用の専用PID。Ideal形式、台形積分・微分フィルター、実測Dt、単精度。  Controller=PID  Form=Ideal  TimeDomain=Discrete-time  UseExternalTs=on  SampleTime=.0025  IntegratorMethod=Trapezoidal  FilterMethod=Trapezoidal  ControllerParametersSource=internal  P=single(0.94999998807907104)  I=single(1)/single(0.69999998807907104)  UseKiTs=off  D=single(0.02500000037252903)  UseExternalDerivativeSource=off  N=single(1)/(single(0.125)*single(0.02500000037252903))  UseFilter=on  TunerSelectOption=Transfer Function Based (PID Tuner App)  InitialConditionSource=external  InitialConditionForIntegrator=0  InitialConditionForFilter=0  DifferentiatorICPrevScaledInput=0  ExternalReset=level  TrackingMode=off  Kt=1  LimitOutput=off  SatLimitsSource=internal  UpperSaturationLimit=inf  LowerSaturationLimit=-inf  LinearizeAsGain=off  AntiWindupMode=none  Kb=1  LimitIntegrator=on  UpperIntegratorSaturationLimit=single(30000)  LowerIntegratorSaturationLimit=single(-30000)  PGainOutDataTypeStr=single  PProdOutDataTypeStr=single  POutMin=[]  POutMax=[]  IGainOutDataTypeStr=single  IProdOutDataTypeStr=single  IOutMin=[]  IOutMax=[]  DGainOutDataTypeStr=single  DProdOutDataTypeStr=single  DOutMin=[]  DOutMax=[]  NGainOutDataTypeStr=single  NProdOutDataTypeStr=single  NOutMin=[]  NOutMax=[]  SumOutDataTypeStr=single  SumOutMin=[]  SumOutMax=[]  SaturationOutDataTypeStr=single  SaturationOutMin=[]  SaturationOutMax=[]  PParamDataTypeStr=single  PParamMin=[]  PParamMax=[]  IParamDataTypeStr=single  IParamMin=[]  IParamMax=[]  DParamDataTypeStr=single  DParamMin=[]  DParamMax=[]  NParamDataTypeStr=single  NParamMin=[]  NParamMax=[]  KbParamDataTypeStr=single  KbParamMin=[]  KbParamMax=[]  KtParamDataTypeStr=single  KtParamMin=[]  KtParamMax=[]  KbOutDataTypeStr=single  KbOutMin=[]  KbOutMax=[]  KtOutDataTypeStr=single  KtOutMin=[]  KtOutMax=[]  IntegratorOutDataTypeStr=single  IntegratorOutMin=[]  IntegratorOutMax=[]  FilterOutDataTypeStr=single  FilterOutMin=[]  FilterOutMax=[]  SumI1OutDataTypeStr=single  SumI1OutMin=[]  SumI1OutMax=[]  SumI2OutDataTypeStr=single  SumI2OutMin=[]  SumI2OutMax=[]  SumI3OutDataTypeStr=single  SumI3OutMin=[]  SumI3OutMax=[]  SumI4OutDataTypeStr=single  SumI4OutMin=[]  SumI4OutMax=[]  SumDOutDataTypeStr=single  SumDOutMin=[]  SumDOutMax=[]  SumAccumDataTypeStr=single  SumI1AccumDataTypeStr=single  SumI2AccumDataTypeStr=single  SumI3AccumDataTypeStr=single  SumI4AccumDataTypeStr=single  SumDAccumDataTypeStr=single  DifferentiatorOutDataTypeStr=single  DifferentiatorOutMin=[]  DifferentiatorOutMax=[]  FilterDiffOutCoefMin=[]  FilterDiffOutCoefMax=[]  ReciprocalOutDataTypeStr=single  ReciprocalOutMin=[]  ReciprocalOutMax=[]  SumDenOutDataTypeStr=single  SumDenOutMin=[]  SumDenOutMax=[]  SumNumOutDataTypeStr=single  SumNumOutMin=[]  SumNumOutMax=[]  SumDenAccumDataTypeStr=single  SumNumAccumDataTypeStr=single  DivideOutDataTypeStr=single  DivideOutMin=[]  DivideOutMax=[]  UdiffTsProdOutDataTypeStr=single  UdiffTsProdOutMin=[]  UdiffTsProdOutMax=[]  NTsProdOutDataTypeStr=single  NTsProdOutMin=[]  NTsProdOutMax=[]  UintegralTsProdOutDataTypeStr=single  UintegralTsProdOutMin=[]  UintegralTsProdOutMax=[]  UngainTsProdOutDataTypeStr=single  UngainTsProdOutMin=[]  UngainTsProdOutMax=[]  ClampingZeroOutDataTypeStr=single  ClampingZeroOutMin=[]  ClampingZeroOutMax=[]  FilterDenConstantOutDataTypeStr=single  FilterDenConstantOutMin=[]  FilterDenConstantOutMax=[]  PCopyOutDataTypeStr=single  PCopyOutMin=[]  PCopyOutMax=[]  NCopyOutDataTypeStr=single  NCopyOutMin=[]  NCopyOutMax=[]  IntegratorContinuousStateAttributes=''  IntegratorStateMustResolveToSignalObject=off  IntegratorRTWStateStorageClass=Auto  FilterContinuousStateAttributes=''  FilterStateMustResolveToSignalObject=off  FilterRTWStateStorageClass=Auto  ParallelPVariant=Passthrough  IdealPVariant=InternalParameters  IVariant=InternalParameters  DVariant=InternalParameters  IntegratorVariant=Discrete  SatVariant=Disabled  AWVariant=Passthrough  PCopyVariant=Disabled  TRVariant=Disabled  FdbkBlocksVariant=Forward  IdealPFdbkVariant=Disabled  SatFdbkVariant=Disabled  DerivativeFilterVariant=TrapezoidalFilter  NVariant=InternalParameters  NCopyVariant=InternalParameters  FilterICVariant=ExternalICs  IntegratorICVariant=ExternalICs  ExternalResetVariant=ExternalReset  TRSumVariant=Passthrough  SumFdbkVariant=Disabled  SumVariant=Sum_PID  TsampFilterVariant=ExternalTs  TsampNgainVariant=Passthrough  TsampIntegralVariant=ExternalTs  ExternalSaturationOutDataTypeStr=Inherit: Same as second input  DerivativeSourceVariant=ErrorSignal  PreIntVariant=InternalPreInt
      settings: LibrarySourceBlock=simulink/Discrete/Discrete PID Controller
  ZeroInitialCondition : Constant  Value=single(0)
  Output : Outport
  wires:
  DedicatedPID/1 -> Output/1
  Reset/1 -> DedicatedPID/2
  Error/1 -> DedicatedPID/1
  Dt/1 -> DedicatedPID/5
  ZeroInitialCondition/1 -> DedicatedPID/3, DedicatedPID/4

== system StampFly_IMU400/FlightControl400/TakeoffHoverControl400/BodyRateControl400/RollRatePID/EnabledPID ==
  Error : Inport
  Dt : Inport  Port=2
  Reset : Inport  Port=3
  Enable : EnablePort
  DedicatedPID : slpidlib/PID Controller  Description=飛行比較用の専用PID。Ideal形式、台形積分・微分フィルター、実測Dt、単精度。  Controller=PID  Form=Ideal  TimeDomain=Discrete-time  UseExternalTs=on  SampleTime=.0025  IntegratorMethod=Trapezoidal  FilterMethod=Trapezoidal  ControllerParametersSource=internal  P=single(0.64999997615814209)  I=single(1)/single(0.69999998807907104)  UseKiTs=off  D=single(0.0099999997764825821)  UseExternalDerivativeSource=off  N=single(1)/(single(0.125)*single(0.0099999997764825821))  UseFilter=on  TunerSelectOption=Transfer Function Based (PID Tuner App)  InitialConditionSource=external  InitialConditionForIntegrator=0  InitialConditionForFilter=0  DifferentiatorICPrevScaledInput=0  ExternalReset=level  TrackingMode=off  Kt=1  LimitOutput=off  SatLimitsSource=internal  UpperSaturationLimit=inf  LowerSaturationLimit=-inf  LinearizeAsGain=off  AntiWindupMode=none  Kb=1  LimitIntegrator=on  UpperIntegratorSaturationLimit=single(30000)  LowerIntegratorSaturationLimit=single(-30000)  PGainOutDataTypeStr=single  PProdOutDataTypeStr=single  POutMin=[]  POutMax=[]  IGainOutDataTypeStr=single  IProdOutDataTypeStr=single  IOutMin=[]  IOutMax=[]  DGainOutDataTypeStr=single  DProdOutDataTypeStr=single  DOutMin=[]  DOutMax=[]  NGainOutDataTypeStr=single  NProdOutDataTypeStr=single  NOutMin=[]  NOutMax=[]  SumOutDataTypeStr=single  SumOutMin=[]  SumOutMax=[]  SaturationOutDataTypeStr=single  SaturationOutMin=[]  SaturationOutMax=[]  PParamDataTypeStr=single  PParamMin=[]  PParamMax=[]  IParamDataTypeStr=single  IParamMin=[]  IParamMax=[]  DParamDataTypeStr=single  DParamMin=[]  DParamMax=[]  NParamDataTypeStr=single  NParamMin=[]  NParamMax=[]  KbParamDataTypeStr=single  KbParamMin=[]  KbParamMax=[]  KtParamDataTypeStr=single  KtParamMin=[]  KtParamMax=[]  KbOutDataTypeStr=single  KbOutMin=[]  KbOutMax=[]  KtOutDataTypeStr=single  KtOutMin=[]  KtOutMax=[]  IntegratorOutDataTypeStr=single  IntegratorOutMin=[]  IntegratorOutMax=[]  FilterOutDataTypeStr=single  FilterOutMin=[]  FilterOutMax=[]  SumI1OutDataTypeStr=single  SumI1OutMin=[]  SumI1OutMax=[]  SumI2OutDataTypeStr=single  SumI2OutMin=[]  SumI2OutMax=[]  SumI3OutDataTypeStr=single  SumI3OutMin=[]  SumI3OutMax=[]  SumI4OutDataTypeStr=single  SumI4OutMin=[]  SumI4OutMax=[]  SumDOutDataTypeStr=single  SumDOutMin=[]  SumDOutMax=[]  SumAccumDataTypeStr=single  SumI1AccumDataTypeStr=single  SumI2AccumDataTypeStr=single  SumI3AccumDataTypeStr=single  SumI4AccumDataTypeStr=single  SumDAccumDataTypeStr=single  DifferentiatorOutDataTypeStr=single  DifferentiatorOutMin=[]  DifferentiatorOutMax=[]  FilterDiffOutCoefMin=[]  FilterDiffOutCoefMax=[]  ReciprocalOutDataTypeStr=single  ReciprocalOutMin=[]  ReciprocalOutMax=[]  SumDenOutDataTypeStr=single  SumDenOutMin=[]  SumDenOutMax=[]  SumNumOutDataTypeStr=single  SumNumOutMin=[]  SumNumOutMax=[]  SumDenAccumDataTypeStr=single  SumNumAccumDataTypeStr=single  DivideOutDataTypeStr=single  DivideOutMin=[]  DivideOutMax=[]  UdiffTsProdOutDataTypeStr=single  UdiffTsProdOutMin=[]  UdiffTsProdOutMax=[]  NTsProdOutDataTypeStr=single  NTsProdOutMin=[]  NTsProdOutMax=[]  UintegralTsProdOutDataTypeStr=single  UintegralTsProdOutMin=[]  UintegralTsProdOutMax=[]  UngainTsProdOutDataTypeStr=single  UngainTsProdOutMin=[]  UngainTsProdOutMax=[]  ClampingZeroOutDataTypeStr=single  ClampingZeroOutMin=[]  ClampingZeroOutMax=[]  FilterDenConstantOutDataTypeStr=single  FilterDenConstantOutMin=[]  FilterDenConstantOutMax=[]  PCopyOutDataTypeStr=single  PCopyOutMin=[]  PCopyOutMax=[]  NCopyOutDataTypeStr=single  NCopyOutMin=[]  NCopyOutMax=[]  IntegratorContinuousStateAttributes=''  IntegratorStateMustResolveToSignalObject=off  IntegratorRTWStateStorageClass=Auto  FilterContinuousStateAttributes=''  FilterStateMustResolveToSignalObject=off  FilterRTWStateStorageClass=Auto  ParallelPVariant=Passthrough  IdealPVariant=InternalParameters  IVariant=InternalParameters  DVariant=InternalParameters  IntegratorVariant=Discrete  SatVariant=Disabled  AWVariant=Passthrough  PCopyVariant=Disabled  TRVariant=Disabled  FdbkBlocksVariant=Forward  IdealPFdbkVariant=Disabled  SatFdbkVariant=Disabled  DerivativeFilterVariant=TrapezoidalFilter  NVariant=InternalParameters  NCopyVariant=InternalParameters  FilterICVariant=ExternalICs  IntegratorICVariant=ExternalICs  ExternalResetVariant=ExternalReset  TRSumVariant=Passthrough  SumFdbkVariant=Disabled  SumVariant=Sum_PID  TsampFilterVariant=ExternalTs  TsampNgainVariant=Passthrough  TsampIntegralVariant=ExternalTs  ExternalSaturationOutDataTypeStr=Inherit: Same as second input  DerivativeSourceVariant=ErrorSignal  PreIntVariant=InternalPreInt
      settings: LibrarySourceBlock=simulink/Discrete/Discrete PID Controller
  ZeroInitialCondition : Constant  Value=single(0)
  Output : Outport
  wires:
  DedicatedPID/1 -> Output/1
  Reset/1 -> DedicatedPID/2
  Error/1 -> DedicatedPID/1
  Dt/1 -> DedicatedPID/5
  ZeroInitialCondition/1 -> DedicatedPID/4, DedicatedPID/3

== system StampFly_IMU400/FlightControl400/TakeoffHoverControl400/BodyRateControl400/YawRatePID/EnabledPID ==
  Error : Inport
  Dt : Inport  Port=2
  Reset : Inport  Port=3
  Enable : EnablePort
  DedicatedPID : slpidlib/PID Controller  Description=飛行比較用の専用PID。Ideal形式、台形積分・微分フィルター、実測Dt、単精度。  Controller=PID  Form=Ideal  TimeDomain=Discrete-time  UseExternalTs=on  SampleTime=.0025  IntegratorMethod=Trapezoidal  FilterMethod=Trapezoidal  ControllerParametersSource=internal  P=single(3)  I=single(1)/single(0.80000001192092896)  UseKiTs=off  D=single(0.0099999997764825821)  UseExternalDerivativeSource=off  N=single(1)/(single(0.125)*single(0.0099999997764825821))  UseFilter=on  TunerSelectOption=Transfer Function Based (PID Tuner App)  InitialConditionSource=external  InitialConditionForIntegrator=0  InitialConditionForFilter=0  DifferentiatorICPrevScaledInput=0  ExternalReset=level  TrackingMode=off  Kt=1  LimitOutput=off  SatLimitsSource=internal  UpperSaturationLimit=inf  LowerSaturationLimit=-inf  LinearizeAsGain=off  AntiWindupMode=none  Kb=1  LimitIntegrator=on  UpperIntegratorSaturationLimit=single(30000)  LowerIntegratorSaturationLimit=single(-30000)  PGainOutDataTypeStr=single  PProdOutDataTypeStr=single  POutMin=[]  POutMax=[]  IGainOutDataTypeStr=single  IProdOutDataTypeStr=single  IOutMin=[]  IOutMax=[]  DGainOutDataTypeStr=single  DProdOutDataTypeStr=single  DOutMin=[]  DOutMax=[]  NGainOutDataTypeStr=single  NProdOutDataTypeStr=single  NOutMin=[]  NOutMax=[]  SumOutDataTypeStr=single  SumOutMin=[]  SumOutMax=[]  SaturationOutDataTypeStr=single  SaturationOutMin=[]  SaturationOutMax=[]  PParamDataTypeStr=single  PParamMin=[]  PParamMax=[]  IParamDataTypeStr=single  IParamMin=[]  IParamMax=[]  DParamDataTypeStr=single  DParamMin=[]  DParamMax=[]  NParamDataTypeStr=single  NParamMin=[]  NParamMax=[]  KbParamDataTypeStr=single  KbParamMin=[]  KbParamMax=[]  KtParamDataTypeStr=single  KtParamMin=[]  KtParamMax=[]  KbOutDataTypeStr=single  KbOutMin=[]  KbOutMax=[]  KtOutDataTypeStr=single  KtOutMin=[]  KtOutMax=[]  IntegratorOutDataTypeStr=single  IntegratorOutMin=[]  IntegratorOutMax=[]  FilterOutDataTypeStr=single  FilterOutMin=[]  FilterOutMax=[]  SumI1OutDataTypeStr=single  SumI1OutMin=[]  SumI1OutMax=[]  SumI2OutDataTypeStr=single  SumI2OutMin=[]  SumI2OutMax=[]  SumI3OutDataTypeStr=single  SumI3OutMin=[]  SumI3OutMax=[]  SumI4OutDataTypeStr=single  SumI4OutMin=[]  SumI4OutMax=[]  SumDOutDataTypeStr=single  SumDOutMin=[]  SumDOutMax=[]  SumAccumDataTypeStr=single  SumI1AccumDataTypeStr=single  SumI2AccumDataTypeStr=single  SumI3AccumDataTypeStr=single  SumI4AccumDataTypeStr=single  SumDAccumDataTypeStr=single  DifferentiatorOutDataTypeStr=single  DifferentiatorOutMin=[]  DifferentiatorOutMax=[]  FilterDiffOutCoefMin=[]  FilterDiffOutCoefMax=[]  ReciprocalOutDataTypeStr=single  ReciprocalOutMin=[]  ReciprocalOutMax=[]  SumDenOutDataTypeStr=single  SumDenOutMin=[]  SumDenOutMax=[]  SumNumOutDataTypeStr=single  SumNumOutMin=[]  SumNumOutMax=[]  SumDenAccumDataTypeStr=single  SumNumAccumDataTypeStr=single  DivideOutDataTypeStr=single  DivideOutMin=[]  DivideOutMax=[]  UdiffTsProdOutDataTypeStr=single  UdiffTsProdOutMin=[]  UdiffTsProdOutMax=[]  NTsProdOutDataTypeStr=single  NTsProdOutMin=[]  NTsProdOutMax=[]  UintegralTsProdOutDataTypeStr=single  UintegralTsProdOutMin=[]  UintegralTsProdOutMax=[]  UngainTsProdOutDataTypeStr=single  UngainTsProdOutMin=[]  UngainTsProdOutMax=[]  ClampingZeroOutDataTypeStr=single  ClampingZeroOutMin=[]  ClampingZeroOutMax=[]  FilterDenConstantOutDataTypeStr=single  FilterDenConstantOutMin=[]  FilterDenConstantOutMax=[]  PCopyOutDataTypeStr=single  PCopyOutMin=[]  PCopyOutMax=[]  NCopyOutDataTypeStr=single  NCopyOutMin=[]  NCopyOutMax=[]  IntegratorContinuousStateAttributes=''  IntegratorStateMustResolveToSignalObject=off  IntegratorRTWStateStorageClass=Auto  FilterContinuousStateAttributes=''  FilterStateMustResolveToSignalObject=off  FilterRTWStateStorageClass=Auto  ParallelPVariant=Passthrough  IdealPVariant=InternalParameters  IVariant=InternalParameters  DVariant=InternalParameters  IntegratorVariant=Discrete  SatVariant=Disabled  AWVariant=Passthrough  PCopyVariant=Disabled  TRVariant=Disabled  FdbkBlocksVariant=Forward  IdealPFdbkVariant=Disabled  SatFdbkVariant=Disabled  DerivativeFilterVariant=TrapezoidalFilter  NVariant=InternalParameters  NCopyVariant=InternalParameters  FilterICVariant=ExternalICs  IntegratorICVariant=ExternalICs  ExternalResetVariant=ExternalReset  TRSumVariant=Passthrough  SumFdbkVariant=Disabled  SumVariant=Sum_PID  TsampFilterVariant=ExternalTs  TsampNgainVariant=Passthrough  TsampIntegralVariant=ExternalTs  ExternalSaturationOutDataTypeStr=Inherit: Same as second input  DerivativeSourceVariant=ErrorSignal  PreIntVariant=InternalPreInt
      settings: LibrarySourceBlock=simulink/Discrete/Discrete PID Controller
  ZeroInitialCondition : Constant  Value=single(0)
  Output : Outport
  wires:
  DedicatedPID/1 -> Output/1
  Reset/1 -> DedicatedPID/2
  Error/1 -> DedicatedPID/1
  Dt/1 -> DedicatedPID/5
  ZeroInitialCondition/1 -> DedicatedPID/3, DedicatedPID/4

== system StampFly_IMU400/FlightControl400/TakeoffHoverControl400/MotorAllocation400/MotorMixerFilter8bit/JapaneseExplanation ==
